simulink model "PV_WIND_BESS_ISLAND_R1"  (R2023b)
settings: Solver=ode14x  StartTime=0.0  StopTime=3.2  FixedStep=25e-6  MaxStep=1e-5  RelTol=1e-3
InitFcn:
  | setup_v2_paths;init_grid_supported_integration;run(which('init_bess_vsm_r10.m'));
undefined symbols (not defined in the file): Base, Control, Converter, DiscIntNeverNeededParam, Drive, Filter, G, PMSG, V2, Wind
libraries: nesl_utility x51, ee_lib x44, fl_lib x25, simulink x6
(part 3 of 4)

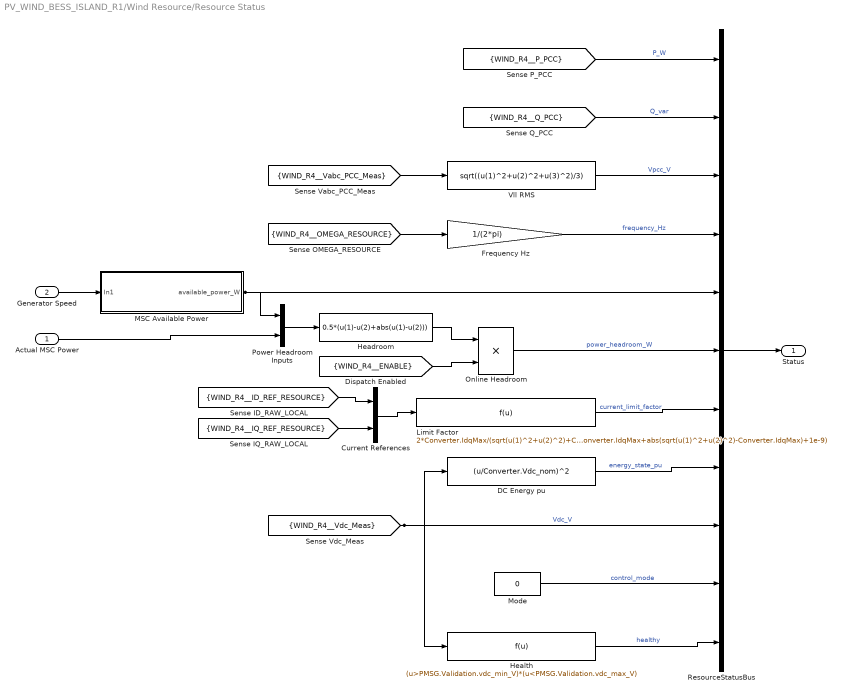
== system PV_WIND_BESS_ISLAND_R1/Wind Resource/Resource Status ==
  Actual MSC Power : Inport
  Generator Speed : Inport  Port=2
  Current References : Mux  Inputs=2
  DC Energy pu : Fcn  Expr=(u/Converter.Vdc_nom)^2
  Frequency Hz : Gain  Gain=1/(2*pi)
  Headroom : Fcn  Expr=0.5*(u(1)-u(2)+abs(u(1)-u(2)))
  Health : Fcn  Expr=(u>PMSG.Validation.vdc_min_V)*(u<PMSG.Validation.vdc_max_V)
  Limit Factor : Fcn  Expr=2*Converter.IdqMax/(sqrt(u(1)^2+u(2)^2)+Converter.IdqMax+abs(sqrt(u(1)^2+u(2)^2)-Converter.IdqMax)+1e-9)
  MSC Available Power : Subsystem
  Mode : Constant  Value=0
  Online Headroom : Product
  Power Headroom Inputs : Mux  Inputs=2
  ResourceStatusBus : BusCreator  Inputs=11  OutDataTypeStr=Bus: ResourceStatusBus
  Vll RMS : Fcn  Expr=sqrt((u(1)^2+u(2)^2+u(3)^2)/3)
  Status : Outport  OutDataTypeStr=Bus: ResourceStatusBus
  wires:
  Generator Speed/1 -> MSC Available Power/1(In1)
  MSC Available Power/1(available_power_W) -> ResourceStatusBus/5, Power Headroom Inputs/1
  ResourceStatusBus/1 -> Status/1
  Health/1 -> ResourceStatusBus/11  "healthy"
  Mode/1 -> ResourceStatusBus/10  "control_mode"
  DC Energy pu/1 -> ResourceStatusBus/8  "energy_state_pu"
  Limit Factor/1 -> ResourceStatusBus/7  "current_limit_factor"
  Online Headroom/1 -> ResourceStatusBus/6  "power_headroom_W"
  Frequency Hz/1 -> ResourceStatusBus/4  "frequency_Hz"
  Vll RMS/1 -> ResourceStatusBus/3  "Vpcc_V"
  [WIND_R4__Q_PCC] -> ResourceStatusBus/2  "Q_var"
  [WIND_R4__P_PCC] -> ResourceStatusBus/1  "P_W"
  [WIND_R4__Vdc_Meas] -> ResourceStatusBus/9, Health/1, DC Energy pu/1  "Vdc_V"
  [WIND_R4__ENABLE] -> Online Headroom/2
  Headroom/1 -> Online Headroom/1
  Power Headroom Inputs/1 -> Headroom/1
  Actual MSC Power/1 -> Power Headroom Inputs/2
  Current References/1 -> Limit Factor/1
  [WIND_R4__IQ_REF_RESOURCE] -> Current References/2
  [WIND_R4__ID_REF_RESOURCE] -> Current References/1
  [WIND_R4__OMEGA_RESOURCE] -> Frequency Hz/1
  [WIND_R4__Vabc_PCC_Meas] -> Vll RMS/1

== system PV_WIND_BESS_ISLAND_R1/02 GFM PCS and Step-up/03 GFM Control and Limits/VSM swing and primary damping ==
  Pcc_W : Inport
  Active command W : Inport  Port=2
  Accelerating power : Sum  Inputs=+-
  Inverse inertia : Gain  Gain=1/(2*G.vsm.H)
  Per unit power : Gain  Gain=1/G.bess.P_W
  Physical RoCoF : Gain  Gain=G.f0_Hz
  Power imbalance W : Sum  Inputs=+-
  Primary damping : Gain  Gain=G.vsm.D
  RoCoF record : ToWorkspace  VariableName=vsm_rocof  SaveFormat=Timeseries  SampleTime=-1
  Rotor speed deviation pu : Integrator
  hertz : Gain  Gain=G.f0_Hz
  rad per second : Gain  Gain=G.w0_rad_s
  deltaOmega : Outport
  deltaHz : Outport  Port=2
  wires:
  Pcc_W/1 -> Power imbalance W/2
  Power imbalance W/1 -> Per unit power/1
  Per unit power/1 -> Accelerating power/1
  Primary damping/1 -> Accelerating power/2
  Accelerating power/1 -> Inverse inertia/1
  Inverse inertia/1 -> Rotor speed deviation pu/1, Physical RoCoF/1
  Rotor speed deviation pu/1 -> Primary damping/1, rad per second/1, hertz/1
  rad per second/1 -> deltaOmega/1
  hertz/1 -> deltaHz/1
  Physical RoCoF/1 -> RoCoF record/1
  Active command W/1 -> Power imbalance W/1

== system PV_WIND_BESS_ISLAND_R1/02 GFM PCS and Step-up/04 PCS Filter and Transformer/Measured voltage and current loops ==
  GFM modulation reference : Inport
  Filter voltage abc : Inport  Port=2
  Inductor current abc : Inport  Port=3
  Grid current abc : Inport  Port=4
  DC volts : Inport  Port=5
  AC waveform record : ToWorkspace  VariableName=r9_feedback  SaveFormat=Timeseries  SampleTime=-1
  Applied modulation record : ToWorkspace  VariableName=r9_modulation  SaveFormat=Timeseries  SampleTime=-1
  Bus voltage ramp : simulink/Sources/Ramp  slope=1/G.vsm.rise_s  start=0  InitialOutput=0
  Cascaded dq regulation : MATLAB Function  TreatAsAtomicUnit=on
  Controller coefficients : Constant  Value=[100e-6;G.filter.L1_H;G.filter.R1_ohm;G.filter.C_F;G.r9.wi;G.r9.wv;G.r9.Ipk;G.dc.modulation_max;G.w0_rad_s]
  Current guard : Constant  Value=G.vsm.guard
  Energization fraction : Saturate  UpperLimit=1  LowerLimit=0
  Feedback vector : Mux  Inputs=5
  Inner loop record : ToWorkspace  VariableName=r9_inner  SaveFormat=Timeseries  SampleTime=-1
  PI states : UnitDelay  InitialCondition=zeros(4,1)  SampleTime=100e-6
  PWM update delay : UnitDelay  InitialCondition=zeros(3,1)  SampleTime=100e-6
  Parallel virtual R and X : Constant  Value=[.16;.16]*G.filter.Zbase_ohm
  Sample feedback : ZeroOrderHold  SampleTime=100e-6
  Sample ramp : ZeroOrderHold  SampleTime=100e-6
  VSM settings : Mux
  modulation : Outport
  wires:
  GFM modulation reference/1 -> Feedback vector/1
  Filter voltage abc/1 -> Feedback vector/2
  Inductor current abc/1 -> Feedback vector/3
  Grid current abc/1 -> Feedback vector/4
  DC volts/1 -> Feedback vector/5
  Feedback vector/1 -> Sample feedback/1
  Sample feedback/1 -> Cascaded dq regulation/1(u), AC waveform record/1
  PI states/1 -> Cascaded dq regulation/2(z)
  Cascaded dq regulation/2(znew) -> PI states/1
  Cascaded dq regulation/1(m) -> PWM update delay/1
  PWM update delay/1 -> modulation/1, Applied modulation record/1
  Cascaded dq regulation/3(diag) -> Inner loop record/1
  Bus voltage ramp/1 -> Energization fraction/1
  Energization fraction/1 -> Sample ramp/1
  Controller coefficients/1 -> VSM settings/1
  Sample ramp/1 -> VSM settings/2
  Current guard/1 -> VSM settings/3
  VSM settings/1 -> Cascaded dq regulation/3(k)
  Parallel virtual R and X/1 -> VSM settings/4

== system PV_WIND_BESS_ISLAND_R1/PV Resource/02 MPPT Boost and DC Link/MPPT and Curtailment ==
  Vpv : Inport
  Ipv : Inport  Port=2
  Vdc : Inport  Port=3
  Command : Inport  Port=4
  01 Sampled PO tracker : Subsystem
  02 Dispatch curtailment : Subsystem
  03 Protected PV target : Subsystem
  04 Boost duty regulator : Subsystem
  PV Power : Product
  Duty : Outport
  Vmp : Outport  Port=2
  Vpv_target : Outport  Port=3
  wires:
  04 Boost duty regulator/1(duty) -> Duty/1
  02 Dispatch curtailment/2(enable) -> 04 Boost duty regulator/3(enable)
  03 Protected PV target/1(target) -> Vpv_target/1, 04 Boost duty regulator/2(target)
  Vdc/1 -> 03 Protected PV target/3(Vdc)
  02 Dispatch curtailment/1(offset) -> 03 Protected PV target/2(offset), 01 Sampled PO tracker/3(Curtailment offset)
  01 Sampled PO tracker/1(Vmp) -> Vmp/1, 03 Protected PV target/1(Vmp)
  Command/1 -> 02 Dispatch curtailment/2(Command)
  PV Power/1 -> 02 Dispatch curtailment/1(Ppv), 01 Sampled PO tracker/2(Ppv)
  Ipv/1 -> PV Power/2
  Vpv/1 -> 04 Boost duty regulator/1(Vpv), 01 Sampled PO tracker/1(Vpv), PV Power/1

== system PV_WIND_BESS_ISLAND_R1/PV Resource/04 Local GFL Control/01 Local PLL ==
  Vabc : Inport
  Angle Integrator : DiscreteIntegrator  InitialCondition=V2.PV.control.pll_theta0_rad  SampleTime=100e-6  ICPrevOutput=DiscIntNeverNeededParam  ICPrevScaledInput=DiscIntNeverNeededParam
  Delta Omega : Sum
  Error Integral : DiscreteIntegrator  SampleTime=100e-6  ICPrevOutput=DiscIntNeverNeededParam  ICPrevScaledInput=DiscIntNeverNeededParam
  Measured Phase : Fcn  Expr=atan2((2/3)*(u(1)-0.5*u(2)-0.5*u(3)),(sqrt(3)/3)*(u(3)-u(2)))
  Nominal Omega : Constant  Value=2*pi*V2.PV.rating.f_Hz
  Omega Command : Sum
  Omega Limits : Saturate  UpperLimit=2*pi*V2.PV.control.pll_max_Hz  LowerLimit=2*pi*V2.PV.control.pll_min_Hz
  PLL Ki : Gain  Gain=V2.PV.control.pll_Ki
  PLL Kp : Gain  Gain=V2.PV.control.pll_Kp
  Phase Pair : Mux  Inputs=2
  Voltage ADC : ZeroOrderHold  SampleTime=100e-6
  Wrapped Phase Error : Fcn  Expr=atan2(sin(u(1)-u(2)),cos(u(1)-u(2)))
  theta : Outport
  omega : Outport  Port=2
  phase_error : Outport  Port=3
  wires:
  Omega Limits/1 -> omega/1, Angle Integrator/1
  Omega Command/1 -> Omega Limits/1
  Nominal Omega/1 -> Omega Command/2
  Delta Omega/1 -> Omega Command/1
  Error Integral/1 -> Delta Omega/2
  PLL Kp/1 -> Delta Omega/1
  PLL Ki/1 -> Error Integral/1
  Wrapped Phase Error/1 -> phase_error/1, PLL Ki/1, PLL Kp/1
  Phase Pair/1 -> Wrapped Phase Error/1
  Angle Integrator/1 -> theta/1, Phase Pair/2
  Measured Phase/1 -> Phase Pair/1
  Vabc/1 -> Voltage ADC/1
  Voltage ADC/1 -> Measured Phase/1

== system PV_WIND_BESS_ISLAND_R1/PV Resource/04 Local GFL Control/02 Measured dq ==
  vabc : Inport
  iabc : Inport  Port=2
  theta : Inport  Port=3
  Id : Fcn  Expr=(2/3)*(u(4)*sin(u(7))+u(5)*sin(u(7)-2*pi/3)+u(6)*sin(u(7)+2*pi/3))
  Iq : Fcn  Expr=(2/3)*(u(4)*cos(u(7))+u(5)*cos(u(7)-2*pi/3)+u(6)*cos(u(7)+2*pi/3))
  Measured abc and Angle : Mux  Inputs=3
  Measured vector : Mux
  Vd : Fcn  Expr=(2/3)*(u(1)*sin(u(7))+u(2)*sin(u(7)-2*pi/3)+u(3)*sin(u(7)+2*pi/3))
  Vq : Fcn  Expr=(2/3)*(u(1)*cos(u(7))+u(2)*cos(u(7)-2*pi/3)+u(3)*cos(u(7)+2*pi/3))
  measured_dq : Outport
  wires:
  Measured vector/1 -> measured_dq/1
  Iq/1 -> Measured vector/4
  Id/1 -> Measured vector/3
  Vq/1 -> Measured vector/2
  Vd/1 -> Measured vector/1
  Measured abc and Angle/1 -> Iq/1, Id/1, Vq/1, Vd/1
  theta/1 -> Measured abc and Angle/3
  iabc/1 -> Measured abc and Angle/2
  vabc/1 -> Measured abc and Angle/1

== system PV_WIND_BESS_ISLAND_R1/PV Resource/04 Local GFL Control/03 Vdc and Q to current reference ==
  measured_dq : Inport
  Vdc : Inport  Port=2
  Ppv : Inport  Port=3
  Command : Inport  Port=4
  Command Selector : BusSelector  OutputSignals=Q_ref_var,enable
  Current Limit Factor : Fcn  Expr=(0.5*((1)+((8135.3825998233579)/(0.5*((sqrt(u(1)^2+u(2)^2))+(1)+abs((sqrt(u(1)^2+u(2)^2))-(1)))))-abs((1)-((8135.3825998233579)/(0.5*((sqrt(u(1)^2+u(2)^2))+(1)+abs((sqrt(u(1)^2+u(2)^2))-(1))))))))
  DC Error : Sum  Inputs=+-
  DC Reference : Constant  Value=V2.PV.dynamic.Vdc_ref_V
  DC Voltage PI : Subsystem
  Enable Ramp : TransferFcn  Numerator=1  Denominator=[V2.PV.dynamic.enable_ramp_s 1]
  Id Limited : Fcn  Expr=u(1)*(0.5*((1)+((8135.3825998233579)/(0.5*((sqrt(u(1)^2+u(2)^2))+(1)+abs((sqrt(u(1)^2+u(2)^2))-(1)))))-abs((1)-((8135.3825998233579)/(0.5*((sqrt(u(1)^2+u(2)^2))+(1)+abs((sqrt(u(1)^2+u(2)^2))-(1))))))))
  Id Unconstrained : Fcn  Expr=(u(2)/(1.5*(0.5*((abs(u(1)))+(200)+abs((abs(u(1)))-(200)))))*u(4)+u(6))*u(5)
  Iq Limited : Fcn  Expr=u(2)*(0.5*((1)+((8135.3825998233579)/(0.5*((sqrt(u(1)^2+u(2)^2))+(1)+abs((sqrt(u(1)^2+u(2)^2))-(1)))))-abs((1)-((8135.3825998233579)/(0.5*((sqrt(u(1)^2+u(2)^2))+(1)+abs((sqrt(u(1)^2+u(2)^2))-(1))))))))
  Iq Unconstrained : Fcn  Expr=-(u(3)-2*pi*(50)*(0.0020893055961443935)*(690)^2)/(1.5*(0.5*((abs(u(1)))+(200)+abs((abs(u(1)))-(200)))))*u(4)*u(5)
  Limited dq : Mux  Inputs=2
  Outer diagnostics : Mux  Inputs=3
  Reference Inputs : Mux  Inputs=6
  Reference Pair : Mux  Inputs=2
  Vd : Fcn  Expr=u(1)
  reference_dq : Outport
  enable : Outport  Port=2
  outer_status : Outport  Port=3
  wires:
  Outer diagnostics/1 -> outer_status/1
  Current Limit Factor/1 -> Outer diagnostics/3
  Limited dq/1 -> reference_dq/1
  Iq Limited/1 -> Limited dq/2
  Id Limited/1 -> Limited dq/1
  Reference Pair/1 -> Iq Limited/1, Id Limited/1, Current Limit Factor/1
  Iq Unconstrained/1 -> Reference Pair/2
  Id Unconstrained/1 -> Reference Pair/1
  Reference Inputs/1 -> Iq Unconstrained/1, Id Unconstrained/1
  DC Voltage PI/1(output) -> Outer diagnostics/1, Reference Inputs/6
  Enable Ramp/1 -> Outer diagnostics/2, Reference Inputs/4
  Command Selector/1 -> Reference Inputs/3  "<Q_ref_var>"
  Ppv/1 -> Reference Inputs/2
  Vd/1 -> Reference Inputs/1
  Command Selector/2 -> enable/1, Reference Inputs/5, Enable Ramp/1  "<enable>"
  Command/1 -> Command Selector/1
  DC Error/1 -> DC Voltage PI/1(error)
  DC Reference/1 -> DC Error/2
  Vdc/1 -> DC Error/1
  measured_dq/1 -> Vd/1

== system PV_WIND_BESS_ISLAND_R1/PV Resource/04 Local GFL Control/04 Current PI and voltage limit ==
  measured_dq : Inport
  reference_dq : Inport  Port=2
  Vdc : Inport  Port=3
  enable : Inport  Port=4
  Applied voltage : Mux  Inputs=2
  Controller Vector : Mux  Inputs=9
  Id Error : Sum  Inputs=+-
  Integral Derivative 1 : Fcn  Expr=(8)*u(1)+(200)*(u(3)-u(5))
  Integral Derivative 2 : Fcn  Expr=(8)*u(2)+(200)*(u(4)-u(6))
  Integral Derivatives : Mux  Inputs=2
  Iq Error : Sum  Inputs=+-
  Measured : Demux
  Reference : Demux  Outputs=2
  Tracking Vector : Mux  Inputs=6
  Vd Applied : Fcn  Expr=u(1)*(0.5*((1)+(((0.97999999999999998)*(0.5*((u(3))+(1)+abs((u(3))-(1))))/2)/(0.5*((sqrt(u(1)^2+u(2)^2))+(1)+abs((sqrt(u(1)^2+u(2)^2))-(1)))))-abs((1)-(((0.97999999999999998)*(0.5*((u(3))+(1)+abs((u(3))-(1))))/2)/(0.5*((sqrt(u(1)^2+u(2)^2))+(1)+abs((sqrt(u(1)^2+u(2)^2))-(1))))))))
  Vd Raw : Fcn  Expr=u(1)+((0.00038088)+(0.00038088))*u(3)-2*pi*(50)*((1.9398059111949151e-05)+(7.2742721669809311e-06))*u(4)+(0.080000000000000002)*u(5)+u(7)
  Voltage Limit Vector : Mux
  Vq Applied : Fcn  Expr=u(2)*(0.5*((1)+(((0.97999999999999998)*(0.5*((u(3))+(1)+abs((u(3))-(1))))/2)/(0.5*((sqrt(u(1)^2+u(2)^2))+(1)+abs((sqrt(u(1)^2+u(2)^2))-(1)))))-abs((1)-(((0.97999999999999998)*(0.5*((u(3))+(1)+abs((u(3))-(1))))/2)/(0.5*((sqrt(u(1)^2+u(2)^2))+(1)+abs((sqrt(u(1)^2+u(2)^2))-(1))))))))
  Vq Raw : Fcn  Expr=u(2)+((0.00038088)+(0.00038088))*u(4)+2*pi*(50)*((1.9398059111949151e-05)+(7.2742721669809311e-06))*u(3)+(0.080000000000000002)*u(6)+u(8)
  dq Integral : DiscreteIntegrator  InitialCondition=[0;0]  SampleTime=100e-6  ICPrevOutput=DiscIntNeverNeededParam  ICPrevScaledInput=DiscIntNeverNeededParam
  voltage_dq : Outport
  wires:
  Applied voltage/1 -> voltage_dq/1
  Integral Derivatives/1 -> dq Integral/1
  Integral Derivative 2/1 -> Integral Derivatives/2
  Integral Derivative 1/1 -> Integral Derivatives/1
  Tracking Vector/1 -> Integral Derivative 2/1, Integral Derivative 1/1
  Vq Applied/1 -> Applied voltage/2, Tracking Vector/4
  Vd Applied/1 -> Applied voltage/1, Tracking Vector/3
  Voltage Limit Vector/1 -> Vq Applied/1, Vd Applied/1
  Vq Raw/1 -> Tracking Vector/6, Voltage Limit Vector/2
  Vd Raw/1 -> Tracking Vector/5, Voltage Limit Vector/1
  Controller Vector/1 -> Vq Raw/1, Vd Raw/1
  enable/1 -> Voltage Limit Vector/4, Controller Vector/9
  Vdc/1 -> Voltage Limit Vector/3, Controller Vector/8
  dq Integral/1 -> Controller Vector/7
  Iq Error/1 -> Tracking Vector/2, Controller Vector/6
  Id Error/1 -> Tracking Vector/1, Controller Vector/5
  Measured/2 -> Controller Vector/2
  Measured/1 -> Controller Vector/1
  Measured/4 -> Controller Vector/4, Iq Error/2
  Reference/2 -> Iq Error/1
  Measured/3 -> Controller Vector/3, Id Error/2
  Reference/1 -> Id Error/1
  reference_dq/1 -> Reference/1
  measured_dq/1 -> Measured/1

== system PV_WIND_BESS_ISLAND_R1/PV Resource/04 Local GFL Control/05 Voltage dq to modulation ==
  voltage_dq : Inport
  theta : Inport  Port=2
  Vdc : Inport  Port=3
  Inverse Park Inputs : Mux  Inputs=3
  Modulation 1 : Fcn  Expr=2*(u(1)*sin(u(3)+(0)*2*pi/3)+u(2)*cos(u(3)+(0)*2*pi/3))/(0.5*((u(4))+(1)+abs((u(4))-(1))))
  Modulation 2 : Fcn  Expr=2*(u(1)*sin(u(3)+(-1)*2*pi/3)+u(2)*cos(u(3)+(-1)*2*pi/3))/(0.5*((u(4))+(1)+abs((u(4))-(1))))
  Modulation 3 : Fcn  Expr=2*(u(1)*sin(u(3)+(-2)*2*pi/3)+u(2)*cos(u(3)+(-2)*2*pi/3))/(0.5*((u(4))+(1)+abs((u(4))-(1))))
  Modulation abc : Mux  Inputs=3
  mabc : Outport
  wires:
  Modulation abc/1 -> mabc/1
  Modulation 3/1 -> Modulation abc/3
  Modulation 2/1 -> Modulation abc/2
  Modulation 1/1 -> Modulation abc/1
  Inverse Park Inputs/1 -> Modulation 3/1, Modulation 2/1, Modulation 1/1
  Vdc/1 -> Inverse Park Inputs/3
  theta/1 -> Inverse Park Inputs/2
  voltage_dq/1 -> Inverse Park Inputs/1

== system PV_WIND_BESS_ISLAND_R1/PV Resource/04 Local GFL Control/06 Control telemetry ==
  reference_dq : Inport
  measured_dq : Inport  Port=2
  outer_status : Inport  Port=3
  Measured : Demux
  Recorder order : Mux  Inputs=6
  Telemetry : Outport
  wires:
  Recorder order/1 -> Telemetry/1
  outer_status/1 -> Recorder order/6
  Measured/2 -> Recorder order/5
  Measured/1 -> Recorder order/4
  Measured/4 -> Recorder order/3
  Measured/3 -> Recorder order/2
  reference_dq/1 -> Recorder order/1
  measured_dq/1 -> Measured/1

== system PV_WIND_BESS_ISLAND_R1/PV Resource/05 Filter Transformer and PCC/PCC Measurement ==
  Local PCC Voltage Record : ToWorkspace  VariableName=pv_v2_pcc_vabc  SampleTime=-1
  Nominal Frequency : Constant  Value=V2.PV.rating.f_Hz
  P to Simulink : nesl_utility/PS-Simulink Converter  PhysicalDomain=network_engine_domain  SubClassName=ps_output  LeftPortType=input  RightPortType=output  PseudoPeriodic=off  Frequencies=[]  VectorFormat=inherit  Unit=W  AffineConversion=off
  PCC Measurement : BusCreator  Inputs=6  OutDataTypeStr=Bus: PCCMeasurementBus
  PCC Power Sensor : ee_lib/Sensors & Transducers/Power Sensor (Three-Phase)  port_option=ee.enum.threePhasePort.composite  load_type=ee.enum.passive.type_balanced.balanced  f0=60 Hz
  PCC VI Sensor : ee_lib/Sensors & Transducers/Current and Voltage Sensor (Three-Phase)  port_option=ee.enum.threePhasePort.composite  vMeasurementType=ee.enum.vmeasurement.ll  outputUnit=ee.enum.unit.si  SRated=100e6 A*V  VRated=24e3 V  I_specify=off  I_priority=None  I=[0, 0, 0] A  I_nominal_specify=off  I_nominal_value=1  I_nominal_unit=A  V_specify=off  V_priority=None  V=[0, 0, 0] V  V_nominal_specify=off  V_nominal_value=1  V_nominal_unit=V
  Q to Simulink : nesl_utility/PS-Simulink Converter  PhysicalDomain=network_engine_domain  SubClassName=ps_output  LeftPortType=input  RightPortType=output  PseudoPeriodic=off  Frequencies=[]  VectorFormat=inherit  Unit=W  AffineConversion=off
  Vll RMS : Fcn  Expr=sqrt((u(1)^2+u(2)^2+u(3)^2)/3)
  iabc to Simulink : nesl_utility/PS-Simulink Converter  PhysicalDomain=network_engine_domain  SubClassName=ps_output  LeftPortType=input  RightPortType=output  PseudoPeriodic=off  Frequencies=[]  VectorFormat=inherit  Unit=A  AffineConversion=off
  vabc to Simulink : nesl_utility/PS-Simulink Converter  PhysicalDomain=network_engine_domain  SubClassName=ps_output  LeftPortType=input  RightPortType=output  PseudoPeriodic=off  Frequencies=[]  VectorFormat=inherit  Unit=V  AffineConversion=off
  From Transformer : PMIOPort  Side=Left  ConnectionType=Connection: foundation.electrical.three_phase
  PCC_10kV : PMIOPort  Port=2  Side=Right  ConnectionType=Connection: foundation.electrical.three_phase
  PCCMeasurementBus : Outport  OutDataTypeStr=Bus: PCCMeasurementBus
  wires:
  PCC Measurement/1 -> PCCMeasurementBus/1
  Nominal Frequency/1 -> PCC Measurement/6  "frequency_Hz"
  Vll RMS/1 -> PCC Measurement/5  "Vll_rms_V"
  Q to Simulink/1 -> PCC Measurement/4  "Q_var"
  P to Simulink/1 -> PCC Measurement/3  "P_W"
  iabc to Simulink/1 -> PCC Measurement/2  "iabc_A"
  vabc to Simulink/1 -> PCC Measurement/1, Vll RMS/1, Local PCC Voltage Record/1  "vabc_V"
  connections:
  PCC Power Sensor/LConn3 -- Q to Simulink/LConn1
  PCC Power Sensor/LConn2 -- P to Simulink/LConn1
  PCC VI Sensor/RConn2 -- iabc to Simulink/LConn1
  PCC VI Sensor/RConn1 -- vabc to Simulink/LConn1
  PCC Power Sensor/RConn1 -- PCC_10kV/RConn1
  PCC VI Sensor/RConn3 -- PCC Power Sensor/LConn1
  From Transformer/RConn1 -- PCC VI Sensor/LConn1

== system PV_WIND_BESS_ISLAND_R1/PV Resource/Resource Status/Commissioning recorder ==
  PCC : Inport
  sourceData : Inport  Port=2
  controlData : Inport  Port=3
  24 channels : Mux  Inputs=5
  Meter : BusSelector  OutputSignals=P_W,Q_var,Vll_rms_V
  Record : ToWorkspace  VariableName=pv_dynamic  SaveFormat=Timeseries  SampleTime=-1
  wires:
  24 channels/1 -> Record/1
  Meter/3 -> 24 channels/5  "<Vll_rms_V>"
  Meter/2 -> 24 channels/4  "<Q_var>"
  Meter/1 -> 24 channels/3  "<P_W>"
  controlData/1 -> 24 channels/2
  sourceData/1 -> 24 channels/1
  PCC/1 -> Meter/1

== system PV_WIND_BESS_ISLAND_R1/PV Resource/Resource Status/DC capability and health ==
  measuredP : Inport
  sourceData : Inport  Port=2
  Available : Constant  Value=V2.PV.rating.P_W*V2.PV.dynamic.irradiance_Wpm2/1000
  Energy : Fcn  Expr=(u/(1500))^2
  Healthy : Fcn  Expr=(u>(900))*(u<(1650))
  Power pair : Mux  Inputs=2
  Reserve : Fcn  Expr=(0.5*((0)+(u(1)-u(2))+abs((0)-(u(1)-u(2)))))
  Vdc : Fcn  Expr=u(3)
  outAvailable : Outport
  outReserve : Outport  Port=2
  outEnergy : Outport  Port=3
  outVdc : Outport  Port=4
  outHealthy : Outport  Port=5
  wires:
  Healthy/1 -> outHealthy/1
  Energy/1 -> outEnergy/1
  Reserve/1 -> outReserve/1
  Vdc/1 -> outVdc/1, Healthy/1, Energy/1
  sourceData/1 -> Vdc/1
  Power pair/1 -> Reserve/1
  measuredP/1 -> Power pair/2
  Available/1 -> outAvailable/1, Power pair/1

== system PV_WIND_BESS_ISLAND_R1/Wind Resource/02 PMSG dq Machine and Average MSC/01 Torque and Current References ==
  omega_g : Inport
  Dispatch Torque Limit : Subsystem
  MPPT Torque Reference : Fcn  Expr=0.5*(Wind.Kopt_Nm_per_rad_s2*u^2+PMSG.torque_limit_Nm-abs(Wind.Kopt_Nm_per_rad_s2*u^2-PMSG.torque_limit_Nm))
  Torque to iq : Gain  Gain=-1/(1.5*PMSG.pole_pairs*PMSG.psi_f_Wb)
  id Reference : Constant  Value=0
  iq Limit : Saturate  UpperLimit=PMSG.current_limit_A  LowerLimit=-PMSG.current_limit_A
  id_ref : Outport
  iq_ref : Outport  Port=2
  wires:
  Dispatch Torque Limit/1(Out1) -> Torque to iq/1
  MPPT Torque Reference/1 -> Dispatch Torque Limit/2(In2)
  omega_g/1 -> MPPT Torque Reference/1, Dispatch Torque Limit/1(In1)
  Torque to iq/1 -> iq Limit/1
  id Reference/1 -> id_ref/1
  iq Limit/1 -> iq_ref/1

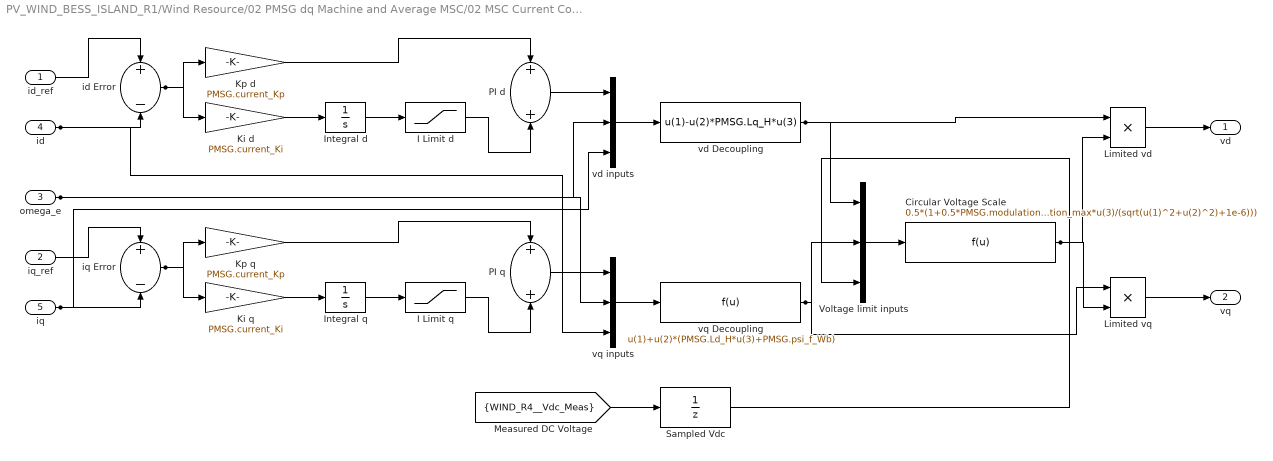
== system PV_WIND_BESS_ISLAND_R1/Wind Resource/02 PMSG dq Machine and Average MSC/02 MSC Current Control ==
  id_ref : Inport
  iq_ref : Inport  Port=2
  omega_e : Inport  Port=3
  id : Inport  Port=4
  iq : Inport  Port=5
  Circular Voltage Scale : Fcn  Expr=0.5*(1+0.5*PMSG.modulation_max*u(3)/(sqrt(u(1)^2+u(2)^2)+1e-6)-abs(1-0.5*PMSG.modulation_max*u(3)/(sqrt(u(1)^2+u(2)^2)+1e-6)))
  I Limit d : Saturate  UpperLimit=PMSG.integrator_limit_V  LowerLimit=-PMSG.integrator_limit_V
  I Limit q : Saturate  UpperLimit=PMSG.integrator_limit_V  LowerLimit=-PMSG.integrator_limit_V
  Integral d : Integrator  InitialCondition=PMSG.Init.vd_pi_V
  Integral q : Integrator  InitialCondition=PMSG.Init.vq_pi_V
  Ki d : Gain  Gain=PMSG.current_Ki
  Ki q : Gain  Gain=PMSG.current_Ki
  Kp d : Gain  Gain=PMSG.current_Kp
  Kp q : Gain  Gain=PMSG.current_Kp
  Limited vd : Product
  Limited vq : Product
  PI d : Sum
  PI q : Sum
  Sampled Vdc : UnitDelay  InitialCondition=Converter.Vdc_nom  SampleTime=100e-6
  Voltage limit inputs : Mux  Inputs=3
  id Error : Sum  Inputs=+-
  iq Error : Sum  Inputs=+-
  vd Decoupling : Fcn  Expr=u(1)-u(2)*PMSG.Lq_H*u(3)
  vd inputs : Mux  Inputs=3
  vq Decoupling : Fcn  Expr=u(1)+u(2)*(PMSG.Ld_H*u(3)+PMSG.psi_f_Wb)
  vq inputs : Mux  Inputs=3
  vd : Outport
  vq : Outport  Port=2
  wires:
  id_ref/1 -> id Error/1
  id/1 -> id Error/2, vq inputs/3
  id Error/1 -> Kp d/1, Ki d/1
  Ki d/1 -> Integral d/1
  Integral d/1 -> I Limit d/1
  Kp d/1 -> PI d/1
  I Limit d/1 -> PI d/2
  PI d/1 -> vd inputs/1
  omega_e/1 -> vd inputs/2, vq inputs/2
  iq/1 -> vd inputs/3, iq Error/2
  vd inputs/1 -> vd Decoupling/1
  iq_ref/1 -> iq Error/1
  iq Error/1 -> Kp q/1, Ki q/1
  Ki q/1 -> Integral q/1
  Integral q/1 -> I Limit q/1
  Kp q/1 -> PI q/1
  I Limit q/1 -> PI q/2
  PI q/1 -> vq inputs/1
  vq inputs/1 -> vq Decoupling/1
  [WIND_R4__Vdc_Meas] -> Sampled Vdc/1
  vd Decoupling/1 -> Voltage limit inputs/1, Limited vd/1
  vq Decoupling/1 -> Voltage limit inputs/2, Limited vq/1
  Sampled Vdc/1 -> Voltage limit inputs/3
  Voltage limit inputs/1 -> Circular Voltage Scale/1
  Circular Voltage Scale/1 -> Limited vd/2, Limited vq/2
  Limited vd/1 -> vd/1
  Limited vq/1 -> vq/1

== system PV_WIND_BESS_ISLAND_R1/Wind Resource/02 PMSG dq Machine and Average MSC/03 PMSG Electrical Dynamics ==
  vd : Inport
  vq : Inport  Port=2
  omega_e : Inport  Port=3
  Electromagnetic Torque : Fcn  Expr=-1.5*PMSG.pole_pairs*(PMSG.psi_f_Wb*u(2)+(PMSG.Ld_H-PMSG.Lq_H)*u(1)*u(2))
  Torque inputs : Mux  Inputs=2
  did dt : Fcn  Expr=(u(1)-PMSG.Rs_ohm*u(2)+u(3)*PMSG.Lq_H*u(4))/PMSG.Ld_H
  did inputs : Mux
  diq dt : Fcn  Expr=(u(1)-PMSG.Rs_ohm*u(2)-u(3)*(PMSG.Ld_H*u(4)+PMSG.psi_f_Wb))/PMSG.Lq_H
  diq inputs : Mux
  id State : Integrator  InitialCondition=PMSG.Init.id_A
  iq State : Integrator  InitialCondition=PMSG.Init.iq_A
  Te : Outport
  id : Outport  Port=2
  iq : Outport  Port=3
  wires:
  vd/1 -> did inputs/1
  id State/1 -> did inputs/2, diq inputs/4, Torque inputs/1, id/1
  omega_e/1 -> did inputs/3, diq inputs/3
  iq State/1 -> did inputs/4, diq inputs/2, Torque inputs/2, iq/1
  did inputs/1 -> did dt/1
  did dt/1 -> id State/1
  vq/1 -> diq inputs/1
  diq inputs/1 -> diq dt/1
  diq dt/1 -> iq State/1
  Torque inputs/1 -> Electromagnetic Torque/1
  Electromagnetic Torque/1 -> Te/1

== system PV_WIND_BESS_ISLAND_R1/Wind Resource/02 PMSG dq Machine and Average MSC/04 MSC DC Power ==
  vd : Inport
  vq : Inport  Port=2
  id : Inport  Port=3
  iq : Inport  Port=4
  Generated DC Power : Fcn  Expr=-1.5*(u(1)*u(3)+u(2)*u(4))*PMSG.msc_efficiency-PMSG.loss_constant_W
  MSC Power Limit : Saturate  UpperLimit=PMSG.Sn_W  LowerLimit=0
  Power inputs : Mux
  Pdc : Outport
  wires:
  vd/1 -> Power inputs/1
  vq/1 -> Power inputs/2
  id/1 -> Power inputs/3
  iq/1 -> Power inputs/4
  Power inputs/1 -> Generated DC Power/1
  Generated DC Power/1 -> MSC Power Limit/1
  MSC Power Limit/1 -> Pdc/1

== system PV_WIND_BESS_ISLAND_R1/Wind Resource/03 DC Link and Two-Level GSC/Converter AC Measurement ==
  note: VSC-side phase voltage, line voltage, and switching current are measured before the RL filter.
  Converter Terminal VI Sensor : ee_lib/Sensors & Transducers/Current and Voltage Sensor (Three-Phase)  port_option=ee.enum.threePhasePort.composite  vMeasurementType=ee.enum.vmeasurement.lg  outputUnit=ee.enum.unit.si  SRated=Base.Sn A*V  VRated=Base.Vll_lv V  I_specify=off  I_priority=None  I=[0, 0, 0] A  I_nominal_specify=off  I_nominal_value=1  I_nominal_unit=A  V_specify=off  V_priority=None  V=[0, 0, 0] V  V_nominal_specify=off  V_nominal_value=1  V_nominal_unit=V
  Iabc to Simulink : nesl_utility/PS-Simulink Converter  PhysicalDomain=network_engine_domain  SubClassName=ps_output  LeftPortType=input  RightPortType=output  PseudoPeriodic=off  Frequencies=[]  VectorFormat=inherit  Unit=A  AffineConversion=off
  Line Voltage Calculation : Subsystem
  Vabc to Simulink : nesl_utility/PS-Simulink Converter  PhysicalDomain=network_engine_domain  SubClassName=ps_output  LeftPortType=input  RightPortType=output  PseudoPeriodic=off  Frequencies=[]  VectorFormat=inherit  Unit=V  AffineConversion=off
  Vll Internal Monitor : Terminator
  From_VSC : PMIOPort  Side=Left
  To_Filter : PMIOPort  Port=2  Side=Right
  tag scope: WIND_R4__Iabc_Converter_Meas=scoped, WIND_R4__Vabc_Converter_Meas=scoped
  wires:
  Vabc to Simulink/1 -> Line Voltage Calculation/1(Vabc), [WIND_R4__Vabc_Converter_Meas]  "Vabc_Converter_Meas"
  Line Voltage Calculation/1(Vll) -> Vll Internal Monitor/1  "Vll_inv"
  Iabc to Simulink/1 -> [WIND_R4__Iabc_Converter_Meas]  "Iabc_Converter_Meas"
  connections:
  From_VSC/RConn1 -- Converter Terminal VI Sensor/LConn1
  Converter Terminal VI Sensor/RConn3 -- To_Filter/RConn1
  Converter Terminal VI Sensor/RConn1 -- Vabc to Simulink/LConn1
  Converter Terminal VI Sensor/RConn2 -- Iabc to Simulink/LConn1

== system PV_WIND_BESS_ISLAND_R1/Wind Resource/03 DC Link and Two-Level GSC/DC Control and Monitoring ==
  note: MSC current command plus two explicit monitor outputs: sampled Vdc and estimated brake current.
  Vdc Measured : Inport
  Pmsc : Inport  Port=2
  Brake Current Estimate : Product
  Brake Current Limit : Saturate  UpperLimit=Wind.brake_current_limit_A  LowerLimit=0
  Brake Hysteresis : Relay  OnSwitchValue=Wind.brake_on_V  OffSwitchValue=Wind.brake_off_V
  Injection Sign : Gain
  MSC Current Inputs : Mux  Inputs=2
  MSC DC Current Limit : Saturate  UpperLimit=Wind.dc_current_limit_A  LowerLimit=0
  Net DC Injection : Sum  Inputs=+-
  P over Vdc : Fcn  Expr=2*u(1)/(u(2)+Wind.dc_voltage_floor_V+abs(u(2)-Wind.dc_voltage_floor_V))
  Sampled DC Voltage : UnitDelay  InitialCondition=Converter.Vdc_nom  SampleTime=100e-6
  Vdc over Brake R : Gain  Gain=1/Wind.brake_R_ohm
  I_msc Command : Outport
  Sampled Vdc : Outport  Port=2
  Brake Current : Outport  Port=3
  tag scope: WIND_R4__Vdc_Meas=scoped
  wires:
  Net DC Injection/1 -> Injection Sign/1
  MSC DC Current Limit/1 -> Net DC Injection/1
  Brake Current Limit/1 -> Net DC Injection/2, Brake Current/1
  Brake Current Estimate/1 -> Brake Current Limit/1
  Pmsc/1 -> MSC Current Inputs/1
  Vdc Measured/1 -> Sampled DC Voltage/1, [WIND_R4__Vdc_Meas]
  Sampled DC Voltage/1 -> Vdc over Brake R/1, Brake Hysteresis/1, MSC Current Inputs/2, Sampled Vdc/1
  MSC Current Inputs/1 -> P over Vdc/1
  P over Vdc/1 -> MSC DC Current Limit/1
  Injection Sign/1 -> I_msc Command/1
  Brake Hysteresis/1 -> Brake Current Estimate/1
  Vdc over Brake R/1 -> Brake Current Estimate/2

== system PV_WIND_BESS_ISLAND_R1/Wind Resource/04 GFL Control and SPWM/01 Measurements and dq ==
  note: Power-invariant Clarke/Park transforms: P = Vd*Id + Vq*Iq; Q = Vq*Id - Vd*Iq.
  Clarke Current : Gain  Gain=sqrt(2/3)*[1 -0.5 -0.5;0 sqrt(3)/2 -sqrt(3)/2]'  Multiplication=Matrix(u*K)
  Clarke Voltage : Gain  Gain=sqrt(2/3)*[1 -0.5 -0.5;0 sqrt(3)/2 -sqrt(3)/2]'  Multiplication=Matrix(u*K)
  Current alpha beta to dq : Subsystem
  Idq Internal Monitor : Terminator
  Instantaneous P : Sum
  Instantaneous Q : Sum  Inputs=+-
  P Internal Monitor : Terminator
  P Low-Pass : TransferFcn  Numerator=[2*pi*Control.Measurement.PowerLPFHz]  Denominator=[1 2*pi*Control.Measurement.PowerLPFHz]
  Q Internal Monitor : Terminator
  Q Low-Pass : TransferFcn  Numerator=[2*pi*Control.Measurement.PowerLPFHz]  Denominator=[1 2*pi*Control.Measurement.PowerLPFHz]
  Separate Idq : Demux  Outputs=2
  Separate Vdq : Demux  Outputs=2
  Vd Id : Product
  Vd Iq : Product
  Vdq Internal Monitor : Terminator
  Voltage alpha beta to dq : Subsystem
  Vq Id : Product
  Vq Iq : Product
  tag scope: WIND_R4__P_PCC=scoped, WIND_R4__Q_PCC=scoped
  wires:
  [WIND_R4__Iabc_PCC_Meas] -> Clarke Current/1
  [WIND_R4__Vabc_PCC_Meas] -> Clarke Voltage/1
  Clarke Current/1 -> Current alpha beta to dq/1(alpha beta)
  [WIND_R4__THETA_PLL_DIAG] -> Current alpha beta to dq/2(theta), Voltage alpha beta to dq/2(theta)
  Current alpha beta to dq/1(dq) -> Idq Internal Monitor/1, Separate Idq/1  "Idq_PCC"
  Vd Id/1 -> Instantaneous P/1
  Vq Iq/1 -> Instantaneous P/2
  Vq Id/1 -> Instantaneous Q/1
  Vd Iq/1 -> Instantaneous Q/2
  P Low-Pass/1 -> [WIND_R4__P_PCC], P Internal Monitor/1  "P_PCC"
  Instantaneous P/1 -> P Low-Pass/1
  Q Low-Pass/1 -> [WIND_R4__Q_PCC], Q Internal Monitor/1  "Q_PCC"
  Instantaneous Q/1 -> Q Low-Pass/1
  Voltage alpha beta to dq/1(dq) -> Separate Vdq/1, Vdq Internal Monitor/1  "Vdq_PCC"
  Separate Vdq/1 -> Vd Id/1, Vd Iq/1
  Separate Idq/1 -> Vd Id/2, Vq Id/2
  Separate Idq/2 -> Vd Iq/2, Vq Iq/2
  Clarke Voltage/1 -> Voltage alpha beta to dq/1(alpha beta)
  Separate Vdq/2 -> Vq Id/1, Vq Iq/1

== system PV_WIND_BESS_ISLAND_R1/Wind Resource/04 GFL Control and SPWM/02 Synchronization SRF-PLL ==
  note: PCC voltage prefilter -> Clarke/Park -> normalized Vq PI -> omega0 bias -> angle integration. Lock target is Vq = 0.
  Angle Integrator : Integrator  InitialCondition=Control.PLL.Theta0
  Clarke abc to alpha beta : Gain  Gain=sqrt(2/3)*[1 -0.5 -0.5;0 sqrt(3)/2 -sqrt(3)/2]'  Multiplication=Matrix(u*K)
  Delta Omega : Sum
  Integrate Vq Error : Integrator
  Nominal Omega : Constant  Value=Control.PLL.OmegaNominal
  Normalize Vq : Gain  Gain=1/Control.PLL.Vbase
  Omega Command : Sum
  Omega Limits : Saturate  UpperLimit=Control.PLL.OmegaMax  LowerLimit=Control.PLL.OmegaMin
  PCC Voltage Prefilter : Subsystem
  PLL Ki : Gain  Gain=Control.PLL.Ki
  PLL Kp : Gain  Gain=Control.PLL.Kp
  Park Voltage : Subsystem
  Separate Vd Vq : Demux  Outputs=2
  Vd PLL Internal Monitor : Terminator
  Vq PLL Internal Monitor : Terminator
  omega Internal Monitor : Terminator
  tag scope: WIND_R4__OMEGA_RESOURCE=scoped, WIND_R4__THETA_PLL_DIAG=scoped
  wires:
  Omega Limits/1 -> [WIND_R4__OMEGA_RESOURCE], Angle Integrator/1, omega Internal Monitor/1  "omega_PLL"
  PCC Voltage Prefilter/1(abc filtered) -> Clarke abc to alpha beta/1
  PLL Kp/1 -> Delta Omega/1
  Integrate Vq Error/1 -> Delta Omega/2
  PLL Ki/1 -> Integrate Vq Error/1
  Separate Vd Vq/2 -> Normalize Vq/1, Vq PLL Internal Monitor/1  "Vq_PLL"
  Nominal Omega/1 -> Omega Command/1
  Delta Omega/1 -> Omega Command/2
  Omega Command/1 -> Omega Limits/1
  [WIND_R4__Vabc_PCC_Meas] -> PCC Voltage Prefilter/1(abc raw)
  Normalize Vq/1 -> PLL Ki/1, PLL Kp/1
  Clarke abc to alpha beta/1 -> Park Voltage/1(alpha beta)
  Angle Integrator/1 -> Park Voltage/2(theta), [WIND_R4__THETA_PLL_DIAG]  "theta_PLL"
  Park Voltage/1(dq) -> Separate Vd Vq/1
  Separate Vd Vq/1 -> Vd PLL Internal Monitor/1  "Vd_PLL"

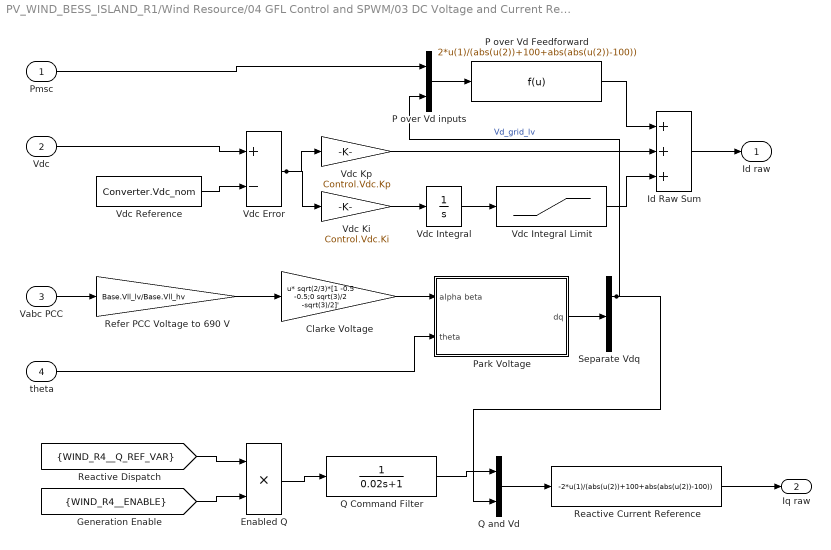
== system PV_WIND_BESS_ISLAND_R1/Wind Resource/04 GFL Control and SPWM/03 DC Voltage and Current Reference ==
  Pmsc : Inport
  Vdc : Inport  Port=2
  Vabc PCC : Inport  Port=3
  theta : Inport  Port=4
  Clarke Voltage : Gain  Gain=sqrt(2/3)*[1 -0.5 -0.5;0 sqrt(3)/2 -sqrt(3)/2]'  Multiplication=Matrix(u*K)
  Enabled Q : Product
  Id Raw Sum : Sum  Inputs=+++
  P over Vd Feedforward : Fcn  Expr=2*u(1)/(abs(u(2))+100+abs(abs(u(2))-100))
  P over Vd inputs : Mux  Inputs=2
  Park Voltage : Subsystem
  Q Command Filter : TransferFcn  Numerator=1  Denominator=[0.02 1]
  Q and Vd : Mux  Inputs=2
  Reactive Current Reference : Fcn  Expr=-2*u(1)/(abs(u(2))+100+abs(abs(u(2))-100))
  Refer PCC Voltage to 690 V : Gain  Gain=Base.Vll_lv/Base.Vll_hv
  Separate Vdq : Demux  Outputs=2
  Vdc Error : Sum  Inputs=+-
  Vdc Integral : Integrator
  Vdc Integral Limit : Saturate  UpperLimit=Control.Vdc.IntegratorLimit  LowerLimit=-Control.Vdc.IntegratorLimit
  Vdc Ki : Gain  Gain=Control.Vdc.Ki
  Vdc Kp : Gain  Gain=Control.Vdc.Kp
  Vdc Reference : Constant  Value=Converter.Vdc_nom
  Id raw : Outport
  Iq raw : Outport  Port=2
  wires:
  Reactive Current Reference/1 -> Iq raw/1
  Q and Vd/1 -> Reactive Current Reference/1
  Q Command Filter/1 -> Q and Vd/1
  Enabled Q/1 -> Q Command Filter/1
  [WIND_R4__ENABLE] -> Enabled Q/2
  [WIND_R4__Q_REF_VAR] -> Enabled Q/1
  Vabc PCC/1 -> Refer PCC Voltage to 690 V/1
  Refer PCC Voltage to 690 V/1 -> Clarke Voltage/1
  Clarke Voltage/1 -> Park Voltage/1(alpha beta)
  theta/1 -> Park Voltage/2(theta)
  Park Voltage/1(dq) -> Separate Vdq/1
  Pmsc/1 -> P over Vd inputs/1
  Separate Vdq/1 -> Q and Vd/2, P over Vd inputs/2  "Vd_grid_lv"
  P over Vd inputs/1 -> P over Vd Feedforward/1
  Vdc/1 -> Vdc Error/1
  Vdc Reference/1 -> Vdc Error/2
  Vdc Error/1 -> Vdc Kp/1, Vdc Ki/1
  Vdc Ki/1 -> Vdc Integral/1
  Vdc Integral/1 -> Vdc Integral Limit/1
  P over Vd Feedforward/1 -> Id Raw Sum/1
  Vdc Kp/1 -> Id Raw Sum/2
  Vdc Integral Limit/1 -> Id Raw Sum/3
  Id Raw Sum/1 -> Id raw/1

== system PV_WIND_BESS_ISLAND_R1/Wind Resource/04 GFL Control and SPWM/04 Circular Current Limiter ==
  note: Circular physical limit preserves dq direction: [Id,Iq]_lim=min(1,Imax/|I*|)[Id,Iq].
  Id raw : Inport
  Iq raw : Inport  Port=2
  Id squared : Product
  Iq squared : Product
  Limit Id : Product
  Limit Iq : Product
  Limiter Active : simulink/Logic and Bit Operations/Compare To Constant  relop=<  const=0.999999  OutDataTypeStr=boolean
  Magnitude : Sqrt
  Magnitude squared : Sum
  Scale factor : Fcn  Expr=0.5*(1+2*Converter.IdqMax/(u+1e-6+abs(u-1e-6))-abs(1-2*Converter.IdqMax/(u+1e-6+abs(u-1e-6))))
  Id limited : Outport
  Iq limited : Outport  Port=2
  Limit active : Outport  Port=3
  tag scope: WIND_R4__ID_REF_RESOURCE=scoped, WIND_R4__IQ_REF_RESOURCE=scoped
  wires:
  Id raw/1 -> [WIND_R4__ID_REF_RESOURCE], Id squared/1, Id squared/2, [WIND_R4__ID_RAW_LOCAL]
  Iq raw/1 -> [WIND_R4__IQ_REF_RESOURCE], Iq squared/1, Iq squared/2, [WIND_R4__IQ_RAW_LOCAL]
  Id squared/1 -> Magnitude squared/1
  Iq squared/1 -> Magnitude squared/2
  Magnitude squared/1 -> Magnitude/1
  Magnitude/1 -> Scale factor/1  "CurrentUtilization"
  [WIND_R4__ID_RAW_LOCAL] -> Limit Id/1
  Scale factor/1 -> Limit Id/2, Limit Iq/1, Limiter Active/1
  [WIND_R4__IQ_RAW_LOCAL] -> Limit Iq/2
  Limit Id/1 -> Id limited/1
  Limit Iq/1 -> Iq limited/1
  Limiter Active/1 -> Limit active/1

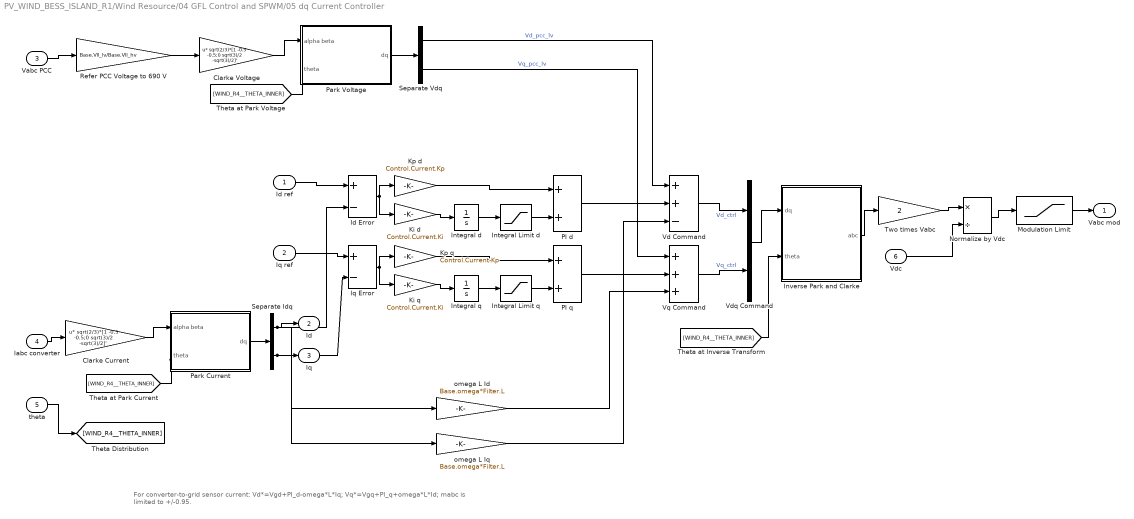
== system PV_WIND_BESS_ISLAND_R1/Wind Resource/04 GFL Control and SPWM/05 dq Current Controller ==
  note: For converter-to-grid sensor current: Vd*=Vgd+PI_d-omega*L*Iq; Vq*=Vgq+PI_q+omega*L*Id; mabc is limited to +/-0.95.
  Id ref : Inport
  Iq ref : Inport  Port=2
  Vabc PCC : Inport  Port=3
  Iabc converter : Inport  Port=4
  theta : Inport  Port=5
  Vdc : Inport  Port=6
  Clarke Current : Gain  Gain=sqrt(2/3)*[1 -0.5 -0.5;0 sqrt(3)/2 -sqrt(3)/2]'  Multiplication=Matrix(u*K)
  Clarke Voltage : Gain  Gain=sqrt(2/3)*[1 -0.5 -0.5;0 sqrt(3)/2 -sqrt(3)/2]'  Multiplication=Matrix(u*K)
  Id Error : Sum  Inputs=+-
  Integral Limit d : Saturate  UpperLimit=Control.Current.IntegratorLimitV  LowerLimit=-Control.Current.IntegratorLimitV
  Integral Limit q : Saturate  UpperLimit=Control.Current.IntegratorLimitV  LowerLimit=-Control.Current.IntegratorLimitV
  Integral d : Integrator
  Integral q : Integrator
  Inverse Park and Clarke : Subsystem
  Iq Error : Sum  Inputs=+-
  Ki d : Gain  Gain=Control.Current.Ki
  Ki q : Gain  Gain=Control.Current.Ki
  Kp d : Gain  Gain=Control.Current.Kp
  Kp q : Gain  Gain=Control.Current.Kp
  Modulation Limit : Saturate  UpperLimit=Converter.ModulationMax  LowerLimit=-Converter.ModulationMax
  Normalize by Vdc : Product  Inputs=*/
  PI d : Sum
  PI q : Sum
  Park Current : Subsystem
  Park Voltage : Subsystem
  Refer PCC Voltage to 690 V : Gain  Gain=Base.Vll_lv/Base.Vll_hv
  Separate Idq : Demux  Outputs=2
  Separate Vdq : Demux  Outputs=2
  Two times Vabc : Gain  Gain=2
  Vd Command : Sum  Inputs=++-
  Vdq Command : Mux  Inputs=2
  Vq Command : Sum  Inputs=+++
  omega L Id : Gain  Gain=Base.omega*Filter.L
  omega L Iq : Gain  Gain=Base.omega*Filter.L
  Vabc mod : Outport
  Id : Outport  Port=2
  Iq : Outport  Port=3
  wires:
  Vabc PCC/1 -> Refer PCC Voltage to 690 V/1
  Refer PCC Voltage to 690 V/1 -> Clarke Voltage/1
  Clarke Voltage/1 -> Park Voltage/1(alpha beta)
  [WIND_R4__THETA_INNER] -> Park Voltage/2(theta)
  Park Voltage/1(dq) -> Separate Vdq/1
  Iabc converter/1 -> Clarke Current/1
  Clarke Current/1 -> Park Current/1(alpha beta)
  [WIND_R4__THETA_INNER] -> Park Current/2(theta)
  Park Current/1(dq) -> Separate Idq/1
  Id ref/1 -> Id Error/1
  Separate Idq/1 -> Id Error/2, omega L Id/1, Id/1
  Iq ref/1 -> Iq Error/1
  Separate Idq/2 -> Iq Error/2, omega L Iq/1, Iq/1
  Id Error/1 -> Kp d/1, Ki d/1
  Ki d/1 -> Integral d/1
  Kp d/1 -> PI d/1
  Integral d/1 -> Integral Limit d/1
  Integral Limit d/1 -> PI d/2
  Iq Error/1 -> Kp q/1, Ki q/1
  Ki q/1 -> Integral q/1
  Kp q/1 -> PI q/1
  Integral q/1 -> Integral Limit q/1
  Integral Limit q/1 -> PI q/2
  Separate Vdq/1 -> Vd Command/1  "Vd_pcc_lv"
  PI d/1 -> Vd Command/2
  omega L Iq/1 -> Vd Command/3
  Separate Vdq/2 -> Vq Command/1  "Vq_pcc_lv"
  PI q/1 -> Vq Command/2
  omega L Id/1 -> Vq Command/3
  Vd Command/1 -> Vdq Command/1  "Vd_ctrl"
  Vq Command/1 -> Vdq Command/2  "Vq_ctrl"
  Vdq Command/1 -> Inverse Park and Clarke/1(dq)
  [WIND_R4__THETA_INNER] -> Inverse Park and Clarke/2(theta)
  theta/1 -> [WIND_R4__THETA_INNER]
  Inverse Park and Clarke/1(abc) -> Two times Vabc/1
  Two times Vabc/1 -> Normalize by Vdc/1
  Vdc/1 -> Normalize by Vdc/2
  Normalize by Vdc/1 -> Modulation Limit/1
  Modulation Limit/1 -> Vabc mod/1

== system PV_WIND_BESS_ISLAND_R1/Wind Resource/04 GFL Control and SPWM/06 Average Duty Interface ==
  note: d_high=(m+1)/2; d_low=1-d_high; output order is [AH AL BH BL CH CL]. One control-step delay is retained.
  Vabc Command : Inport
  A Duty Negate : Gain  Gain=-1
  A Low Duty : Bias  Bias=1  SaturateOnIntegerOverflow=off
  B Duty Negate : Gain  Gain=-1
  B Low Duty : Bias  Bias=1  SaturateOnIntegerOverflow=off
  C Duty Negate : Gain  Gain=-1
  C Low Duty : Bias  Bias=1  SaturateOnIntegerOverflow=off
  Duty 1 to Physical : nesl_utility/Simulink-PS Converter  PhysicalDomain=network_engine_domain  SubClassName=ps_input  LeftPortType=input  RightPortType=output  PseudoPeriodic=off  Frequencies=[]  NoiseDistribution=none  NoiseParameters=[]  Unit=V  AffineConversion=off  FilteringAndDerivatives=provide  SimscapeFilterOrder=1  InputFilterTimeConstant=0.001  UdotUserProvided=0
  Duty 2 to Physical : nesl_utility/Simulink-PS Converter  PhysicalDomain=network_engine_domain  SubClassName=ps_input  LeftPortType=input  RightPortType=output  PseudoPeriodic=off  Frequencies=[]  NoiseDistribution=none  NoiseParameters=[]  Unit=V  AffineConversion=off  FilteringAndDerivatives=provide  SimscapeFilterOrder=1  InputFilterTimeConstant=0.001  UdotUserProvided=0
  Duty 3 to Physical : nesl_utility/Simulink-PS Converter  PhysicalDomain=network_engine_domain  SubClassName=ps_input  LeftPortType=input  RightPortType=output  PseudoPeriodic=off  Frequencies=[]  NoiseDistribution=none  NoiseParameters=[]  Unit=V  AffineConversion=off  FilteringAndDerivatives=provide  SimscapeFilterOrder=1  InputFilterTimeConstant=0.001  UdotUserProvided=0
  Duty 4 to Physical : nesl_utility/Simulink-PS Converter  PhysicalDomain=network_engine_domain  SubClassName=ps_input  LeftPortType=input  RightPortType=output  PseudoPeriodic=off  Frequencies=[]  NoiseDistribution=none  NoiseParameters=[]  Unit=V  AffineConversion=off  FilteringAndDerivatives=provide  SimscapeFilterOrder=1  InputFilterTimeConstant=0.001  UdotUserProvided=0
  Duty 5 to Physical : nesl_utility/Simulink-PS Converter  PhysicalDomain=network_engine_domain  SubClassName=ps_input  LeftPortType=input  RightPortType=output  PseudoPeriodic=off  Frequencies=[]  NoiseDistribution=none  NoiseParameters=[]  Unit=V  AffineConversion=off  FilteringAndDerivatives=provide  SimscapeFilterOrder=1  InputFilterTimeConstant=0.001  UdotUserProvided=0
  Duty 6 to Physical : nesl_utility/Simulink-PS Converter  PhysicalDomain=network_engine_domain  SubClassName=ps_input  LeftPortType=input  RightPortType=output  PseudoPeriodic=off  Frequencies=[]  NoiseDistribution=none  NoiseParameters=[]  Unit=V  AffineConversion=off  FilteringAndDerivatives=provide  SimscapeFilterOrder=1  InputFilterTimeConstant=0.001  UdotUserProvided=0
  Half Modulation : Gain  Gain=0.5
  High-Side Duty : Bias  Bias=0.5  SaturateOnIntegerOverflow=off
  Modulation Limit : Saturate  UpperLimit=Converter.ModulationMax  LowerLimit=-Converter.ModulationMax
  One Control-Step Delay : UnitDelay  InitialCondition=[0 0 0]  SampleTime=100e-6
  Phase Duty Selector : Demux  Outputs=3
  Six-Pulse Duty Multiplexer : ee_lib/Semiconductors & Converters/Converters/Six-Pulse Gate Multiplexer  port_option=ee.enum.controlport.ps
  Duty6 : PMIOPort  Side=Right
  wires:
  Vabc Command/1 -> One Control-Step Delay/1
  One Control-Step Delay/1 -> Modulation Limit/1
  Modulation Limit/1 -> Half Modulation/1
  Half Modulation/1 -> High-Side Duty/1
  High-Side Duty/1 -> Phase Duty Selector/1
  Phase Duty Selector/1 -> Duty 1 to Physical/1, A Duty Negate/1
  A Duty Negate/1 -> A Low Duty/1
  A Low Duty/1 -> Duty 2 to Physical/1
  Phase Duty Selector/2 -> Duty 3 to Physical/1, B Duty Negate/1
  B Duty Negate/1 -> B Low Duty/1
  B Low Duty/1 -> Duty 4 to Physical/1
  Phase Duty Selector/3 -> Duty 5 to Physical/1, C Duty Negate/1
  C Duty Negate/1 -> C Low Duty/1
  C Low Duty/1 -> Duty 6 to Physical/1
  connections:
  Duty 1 to Physical/RConn1 -- Six-Pulse Duty Multiplexer/LConn1
  Duty 2 to Physical/RConn1 -- Six-Pulse Duty Multiplexer/LConn2
  Duty 3 to Physical/RConn1 -- Six-Pulse Duty Multiplexer/LConn3
  Duty 4 to Physical/RConn1 -- Six-Pulse Duty Multiplexer/LConn4
  Duty 5 to Physical/RConn1 -- Six-Pulse Duty Multiplexer/LConn5
  Duty 6 to Physical/RConn1 -- Six-Pulse Duty Multiplexer/LConn6
  Six-Pulse Duty Multiplexer/RConn1 -- Duty6/RConn1

== system PV_WIND_BESS_ISLAND_R1/Wind Resource/Resource Status/MSC Available Power ==
  In1 : Inport
  Available Airgap Power : Product
  Available Auxiliary Loss : Bias  Bias=-PMSG.loss_constant_W  SaturateOnIntegerOverflow=off
  Available MPPT Torque : Fcn  Expr=0.5*(Wind.Kopt_Nm_per_rad_s2*u^2+PMSG.torque_limit_Nm-abs(Wind.Kopt_Nm_per_rad_s2*u^2-PMSG.torque_limit_Nm))
  Available MSC Efficiency : Gain  Gain=PMSG.msc_efficiency
  Available Machine Power : Sum  Inputs=+-
  Available Power Limit : Saturate  UpperLimit=PMSG.Sn_W  LowerLimit=0
  Available iq : Gain  Gain=-1/(1.5*PMSG.pole_pairs*PMSG.psi_f_Wb)
  Available iq squared : Product
  Estimated Copper Loss : Gain  Gain=1.5*PMSG.Rs_ohm
  available_power_W : Outport
  wires:
  Available iq/1 -> Available iq squared/2, Available iq squared/1
  Available Airgap Power/1 -> Available Machine Power/1
  Available Machine Power/1 -> Available MSC Efficiency/1
  Available MPPT Torque/1 -> Available iq/1, Available Airgap Power/1
  In1/1 -> Available Airgap Power/2, Available MPPT Torque/1
  Available Auxiliary Loss/1 -> Available Power Limit/1
  Available iq squared/1 -> Estimated Copper Loss/1
  Available Power Limit/1 -> available_power_W/1  "available_power_W"
  Available MSC Efficiency/1 -> Available Auxiliary Loss/1
  Estimated Copper Loss/1 -> Available Machine Power/2

== system PV_WIND_BESS_ISLAND_R1/PV Resource/02 MPPT Boost and DC Link/MPPT and Curtailment/01 Sampled PO tracker ==
  Vpv : Inport
  Ppv : Inport  Port=2
  Curtailment offset : Inport  Port=3
  Authorized perturbation : Product
  Delta Power : Sum  Inputs=+-
  Delta Voltage : Sum  Inputs=+-
  Gradient Pair : Mux  Inputs=2
  MPPT Voltage : DiscreteIntegrator  IntegratorMethod=Accumulation: Forward Euler  gainval=1  InitialCondition=V2.PV.dynamic.Vmp_initial_V  SampleTime=V2.PV.dynamic.mppt_period_s  LimitOutput=on  UpperSaturationLimit=970  LowerSaturationLimit=V2.PV.dynamic.Vpv_min_V  ICPrevOutput=DiscIntNeverNeededParam  ICPrevScaledInput=DiscIntNeverNeededParam
  MPPT active : simulink/Logic and Bit Operations/Compare To Constant  relop=<=  const=V2.PV.dynamic.mppt_step_V  OutDataTypeStr=boolean
  PO Direction : Fcn  Expr=2*(u(1)*u(2)>=0)-1
  PO Step : Gain  Gain=V2.PV.dynamic.mppt_step_V
  Previous Power : UnitDelay  SampleTime=V2.PV.dynamic.mppt_period_s
  Previous Voltage : UnitDelay  InitialCondition=V2.PV.dynamic.Vmp_initial_V  SampleTime=V2.PV.dynamic.mppt_period_s
  Sample Power : ZeroOrderHold  SampleTime=V2.PV.dynamic.mppt_period_s
  Sample Voltage : ZeroOrderHold  SampleTime=V2.PV.dynamic.mppt_period_s
  Sample offset : ZeroOrderHold  SampleTime=V2.PV.dynamic.mppt_period_s
  Vmp : Outport
  wires:
  MPPT Voltage/1 -> Vmp/1
  PO Direction/1 -> PO Step/1
  Gradient Pair/1 -> PO Direction/1
  Delta Power/1 -> Gradient Pair/2
  Delta Voltage/1 -> Gradient Pair/1
  Previous Power/1 -> Delta Power/2
  Previous Voltage/1 -> Delta Voltage/2
  Sample Power/1 -> Delta Power/1, Previous Power/1
  Sample Voltage/1 -> Delta Voltage/1, Previous Voltage/1
  Ppv/1 -> Sample Power/1
  Vpv/1 -> Sample Voltage/1
  Curtailment offset/1 -> Sample offset/1
  Sample offset/1 -> MPPT active/1
  MPPT active/1 -> Authorized perturbation/2
  PO Step/1 -> Authorized perturbation/1
  Authorized perturbation/1 -> MPPT Voltage/1

== system PV_WIND_BESS_ISLAND_R1/PV Resource/02 MPPT Boost and DC Link/MPPT and Curtailment/02 Dispatch curtailment ==
  Ppv : Inport
  Command : Inport  Port=2
  Command Selector : BusSelector  OutputSignals=P_ref_W,enable
  Curtailment Error : Sum  Inputs=+-
  Curtailment PI : Subsystem
  Dispatch Limit : Saturate  UpperLimit=V2.PV.rating.P_W  LowerLimit=0
  Enabled Dispatch : Product
  offset : Outport
  enable : Outport  Port=2
  wires:
  Curtailment PI/1(output) -> offset/1
  Curtailment Error/1 -> Curtailment PI/1(error)
  Enabled Dispatch/1 -> Curtailment Error/2
  Ppv/1 -> Curtailment Error/1
  Command Selector/2 -> enable/1, Enabled Dispatch/2  "<enable>"
  Dispatch Limit/1 -> Enabled Dispatch/1
  Command Selector/1 -> Dispatch Limit/1  "<P_ref_W>"
  Command/1 -> Command Selector/1

== system PV_WIND_BESS_ISLAND_R1/PV Resource/02 MPPT Boost and DC Link/MPPT and Curtailment/03 Protected PV target ==
  Vmp : Inport
  offset : Inport  Port=2
  Vdc : Inport  Port=3
  DC Overvoltage Curtailment : Fcn  Expr=u(1)+2*(0.5*((0)+(u(2)-(1650))+abs((0)-(u(2)-(1650)))))
  Overvoltage Inputs : Mux  Inputs=2
  PV Target Limit : Saturate  UpperLimit=V2.PV.dynamic.Vpv_max_V  LowerLimit=V2.PV.dynamic.Vpv_min_V
  Voltage Target : Sum
  target : Outport
  wires:
  PV Target Limit/1 -> target/1
  DC Overvoltage Curtailment/1 -> PV Target Limit/1
  Overvoltage Inputs/1 -> DC Overvoltage Curtailment/1
  Vdc/1 -> Overvoltage Inputs/2
  Voltage Target/1 -> Overvoltage Inputs/1
  offset/1 -> Voltage Target/2
  Vmp/1 -> Voltage Target/1

== system PV_WIND_BESS_ISLAND_R1/PV Resource/02 MPPT Boost and DC Link/MPPT and Curtailment/04 Boost duty regulator ==
  Vpv : Inport
  target : Inport  Port=2
  enable : Inport  Port=3
  Boost Voltage Error : Sum  Inputs=+-
  Boost Voltage PI : Subsystem
  Enable Boost : Product
  duty : Outport
  wires:
  Enable Boost/1 -> duty/1
  enable/1 -> Enable Boost/2
  Boost Voltage PI/1(output) -> Enable Boost/1
  Boost Voltage Error/1 -> Boost Voltage PI/1(error)
  target/1 -> Boost Voltage Error/2
  Vpv/1 -> Boost Voltage Error/1
